simulink model "lab09_observer_controller"  (R2026b)
settings: Solver=VariableStepAuto  StopTime=1.5  RelTol=1e-9
undefined symbols (not defined in the file): A_o, B_o, C_o, D_o, Ki_cont, Km, Kp, tau, Ts, Vdc
libraries: slpidlib x3
settings Model: Creator=Maddo  LastModifiedBy=Maddo
settings DataIOCC: SaveFormat=Structure

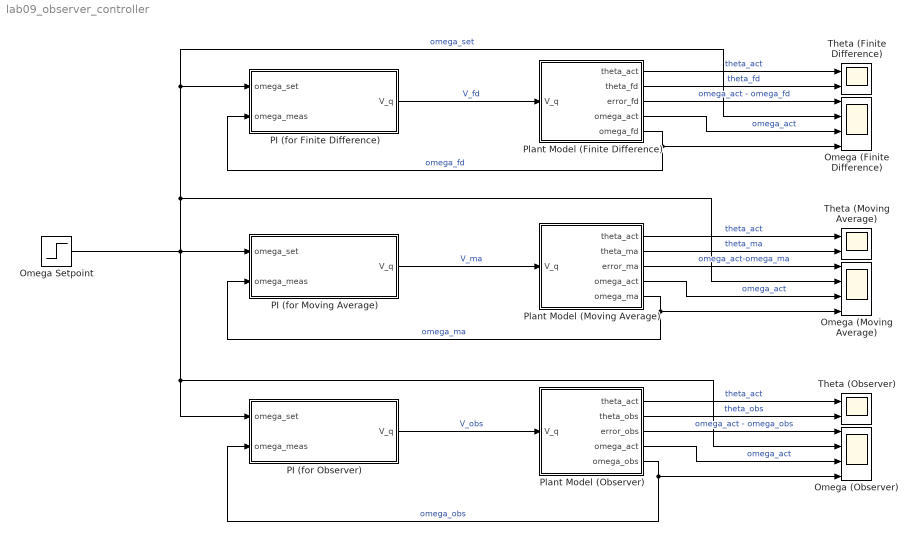
== system lab09_observer_controller ==
  Omega (Finite Difference) : Scope  NumInputPorts=4
      settings: ActiveDisplayYMinimum=-0.40086586035071825  ActiveDisplayYMaximum=0.41815649863978394  DataLoggingVariableName=ScopeData7
  Omega (Moving Average) : Scope  NumInputPorts=4
      settings: ActiveDisplayYMinimum=-1  ActiveDisplayYMaximum=1
  Omega (Observer) : Scope  NumInputPorts=4
      settings: ActiveDisplayYMinimum=-0.10732048180331535  ActiveDisplayYMaximum=0.23324163544595725  DataLoggingVariableName=ScopeData4
  Omega Setpoint : Step  Time=0  FinalValue=omega_set  SampleTime=0
  PI (for Finite Difference) : Subsystem
  PI (for Moving Average) : Subsystem
  PI (for Observer) : Subsystem
  Plant Model (Finite Difference) : Subsystem
  Plant Model (Moving Average) : Subsystem
  Plant Model (Observer) : Subsystem
  Theta (Finite Difference) : Scope  NumInputPorts=2
      settings: ActiveDisplayYMinimum=-1  ActiveDisplayYMaximum=1
  Theta (Moving Average) : Scope  NumInputPorts=2
      settings: ActiveDisplayYMinimum=-1  ActiveDisplayYMaximum=1  DataLoggingVariableName=ScopeData2
  Theta (Observer) : Scope  NumInputPorts=2
      settings: ActiveDisplayYMinimum=1.7677662447249645  ActiveDisplayYMaximum=1.9037236023326192  DataLoggingVariableName=ScopeData5
  wires:
  Plant Model (Finite Difference)/1(theta_act) -> Theta (Finite Difference)/1  "theta_act"
  Plant Model (Finite Difference)/2(theta_fd) -> Theta (Finite Difference)/2  "theta_fd"
  Plant Model (Finite Difference)/4(omega_act) -> Omega (Finite Difference)/3  "omega_act"
  Plant Model (Finite Difference)/5(omega_fd) -> PI (for Finite Difference)/2(omega_meas), Omega (Finite Difference)/4  "omega_fd"
  Plant Model (Finite Difference)/3(error_fd) -> Omega (Finite Difference)/1  "omega_act - omega_fd"
  Plant Model (Moving Average)/3(error_ma) -> Omega (Moving Average)/1  "omega_act-omega_ma"
  Plant Model (Moving Average)/5(omega_ma) -> PI (for Moving Average)/2(omega_meas), Omega (Moving Average)/4  "omega_ma"
  Plant Model (Moving Average)/4(omega_act) -> Omega (Moving Average)/3  "omega_act"
  Plant Model (Moving Average)/2(theta_ma) -> Theta (Moving Average)/2  "theta_ma"
  Plant Model (Moving Average)/1(theta_act) -> Theta (Moving Average)/1  "theta_act"
  Plant Model (Observer)/1(theta_act) -> Theta (Observer)/1  "theta_act"
  Plant Model (Observer)/2(theta_obs) -> Theta (Observer)/2  "theta_obs"
  Plant Model (Observer)/4(omega_act) -> Omega (Observer)/3  "omega_act"
  Plant Model (Observer)/5(omega_obs) -> PI (for Observer)/2(omega_meas), Omega (Observer)/4  "omega_obs"
  Plant Model (Observer)/3(error_obs) -> Omega (Observer)/1  "omega_act - omega_obs"
  Omega Setpoint/1 -> Omega (Moving Average)/2, Omega (Finite Difference)/2, PI (for Finite Difference)/1(omega_set), PI (for Moving Average)/1(omega_set), PI (for Observer)/1(omega_set), Omega (Observer)/2  "omega_set"
  PI (for Finite Difference)/1(V_q) -> Plant Model (Finite Difference)/1(V_q)  "V_fd"
  PI (for Moving Average)/1(V_q) -> Plant Model (Moving Average)/1(V_q)  "V_ma"
  PI (for Observer)/1(V_q) -> Plant Model (Observer)/1(V_q)  "V_obs"

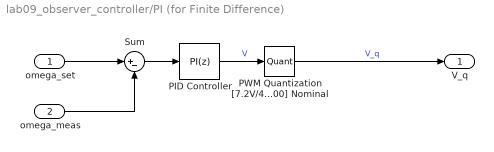
== system lab09_observer_controller/PI (for Finite Difference) ==
  omega_set : Inport
  omega_meas : Inport  Port=2
  PID Controller : slpidlib/PID Controller  Controller=PI  Form=Parallel  TimeDomain=Discrete-time  UseExternalTs=off  SampleTime=Ts  IntegratorMethod=Forward Euler  FilterMethod=Forward Euler  ControllerParametersSource=internal  P=Kp  I=Ki_cont  UseKiTs=off  D=0  UseExternalDerivativeSource=off  N=100  UseFilter=on  TunerSelectOption=Transfer Function Based (PID Tuner App)  InitialConditionSource=internal  InitialConditionForIntegrator=0  InitialConditionForFilter=0  DifferentiatorICPrevScaledInput=0  ExternalReset=none  TrackingMode=off  Kt=1  LimitOutput=on  SatLimitsSource=internal  UpperSaturationLimit=Vdc  LowerSaturationLimit=-Vdc  LinearizeAsGain=on  AntiWindupMode=clamping  Kb=1  LimitIntegrator=off  UpperIntegratorSaturationLimit=inf  LowerIntegratorSaturationLimit=-inf  POutMin=[]  POutMax=[]  IOutMin=[]  IOutMax=[]  DOutMin=[]  DOutMax=[]  NOutMin=[]  NOutMax=[]  SumOutMin=[]  SumOutMax=[]  SaturationOutMin=[]  SaturationOutMax=[]  PParamMin=[]  PParamMax=[]  IParamMin=[]  IParamMax=[]  DParamMin=[]  DParamMax=[]  NParamMin=[]  NParamMax=[]  KbParamMin=[]  KbParamMax=[]  KtParamMin=[]  KtParamMax=[]  KbOutMin=[]  KbOutMax=[]  KtOutMin=[]  KtOutMax=[]  IntegratorOutMin=[]  IntegratorOutMax=[]  FilterOutMin=[]  FilterOutMax=[]  SumI1OutMin=[]  SumI1OutMax=[]  SumI2OutMin=[]  SumI2OutMax=[]  SumI3OutMin=[]  SumI3OutMax=[]  SumI4OutMin=[]  SumI4OutMax=[]  SumDOutMin=[]  SumDOutMax=[]  DifferentiatorOutMin=[]  DifferentiatorOutMax=[]  FilterDiffOutCoefMin=[]  FilterDiffOutCoefMax=[]  ReciprocalOutMin=[]  ReciprocalOutMax=[]  SumDenOutMin=[]  SumDenOutMax=[]  SumNumOutMin=[]  SumNumOutMax=[]  DivideOutMin=[]  DivideOutMax=[]  UdiffTsProdOutMin=[]  UdiffTsProdOutMax=[]  NTsProdOutMin=[]  NTsProdOutMax=[]  UintegralTsProdOutMin=[]  UintegralTsProdOutMax=[]  UngainTsProdOutMin=[]  UngainTsProdOutMax=[]  ClampingZeroOutDataTypeStr=Inherit: Inherit via back propagation  ClampingZeroOutMin=[]  ClampingZeroOutMax=[]  FilterDenConstantOutDataTypeStr=Inherit: Inherit via back propagation  FilterDenConstantOutMin=[]  FilterDenConstantOutMax=[]  PCopyOutDataTypeStr=Inherit: Inherit via back propagation  PCopyOutMin=[]  PCopyOutMax=[]  NCopyOutDataTypeStr=Inherit: Inherit via back propagation  NCopyOutMin=[]  NCopyOutMax=[]  IntegratorContinuousStateAttributes=''  IntegratorStateMustResolveToSignalObject=off  IntegratorRTWStateStorageClass=Auto  FilterContinuousStateAttributes=''  FilterStateMustResolveToSignalObject=off  FilterRTWStateStorageClass=Auto  ParallelPVariant=InternalParameters  IdealPVariant=Disabled  IVariant=InternalParameters  DVariant=Disabled  IntegratorVariant=Discrete  SatVariant=Enabled  AWVariant=DiscClampingParallel  PCopyVariant=Disabled  TRVariant=Disabled  FdbkBlocksVariant=Forward  IdealPFdbkVariant=Disabled  SatFdbkVariant=Disabled  DerivativeFilterVariant=Disabled  NVariant=Disabled  NCopyVariant=Disabled_SignalSpec  FilterICVariant=Disabled  IntegratorICVariant=InternalICs  ExternalResetVariant=Disabled  TRSumVariant=Passthrough  SumFdbkVariant=Disabled  SumVariant=Sum_PI  TsampFilterVariant=InternalTs  TsampNgainVariant=Passthrough  TsampIntegralVariant=Disabled_SignalSpec  ExternalSaturationOutDataTypeStr=Inherit: Same as second input  DerivativeSourceVariant=Disabled  PreIntVariant=InternalPreInt
  PWM Quantization [7.2V/4000] Nominal : Quantizer  QuantizationInterval=Vdc/4000
  Sum : Sum  Inputs=|+-
  V_q : Outport
  wires:
  Sum/1 -> PID Controller/1
  PWM Quantization [7.2V/4000] Nominal/1 -> V_q/1  "V_q"
  PID Controller/1 -> PWM Quantization [7.2V/4000] Nominal/1  "V"
  omega_set/1 -> Sum/1
  omega_meas/1 -> Sum/2

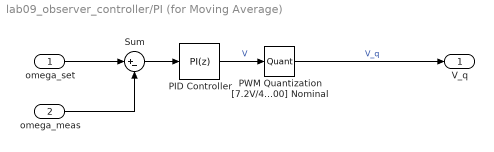
== system lab09_observer_controller/PI (for Moving Average) ==
  omega_set : Inport
  omega_meas : Inport  Port=2
  PID Controller : slpidlib/PID Controller  Controller=PI  Form=Parallel  TimeDomain=Discrete-time  UseExternalTs=off  SampleTime=Ts  IntegratorMethod=Forward Euler  FilterMethod=Forward Euler  ControllerParametersSource=internal  P=Kp  I=Ki_cont  UseKiTs=off  D=0  UseExternalDerivativeSource=off  N=100  UseFilter=on  TunerSelectOption=Transfer Function Based (PID Tuner App)  InitialConditionSource=internal  InitialConditionForIntegrator=0  InitialConditionForFilter=0  DifferentiatorICPrevScaledInput=0  ExternalReset=none  TrackingMode=off  Kt=1  LimitOutput=on  SatLimitsSource=internal  UpperSaturationLimit=Vdc  LowerSaturationLimit=-Vdc  LinearizeAsGain=on  AntiWindupMode=clamping  Kb=1  LimitIntegrator=off  UpperIntegratorSaturationLimit=inf  LowerIntegratorSaturationLimit=-inf  POutMin=[]  POutMax=[]  IOutMin=[]  IOutMax=[]  DOutMin=[]  DOutMax=[]  NOutMin=[]  NOutMax=[]  SumOutMin=[]  SumOutMax=[]  SaturationOutMin=[]  SaturationOutMax=[]  PParamMin=[]  PParamMax=[]  IParamMin=[]  IParamMax=[]  DParamMin=[]  DParamMax=[]  NParamMin=[]  NParamMax=[]  KbParamMin=[]  KbParamMax=[]  KtParamMin=[]  KtParamMax=[]  KbOutMin=[]  KbOutMax=[]  KtOutMin=[]  KtOutMax=[]  IntegratorOutMin=[]  IntegratorOutMax=[]  FilterOutMin=[]  FilterOutMax=[]  SumI1OutMin=[]  SumI1OutMax=[]  SumI2OutMin=[]  SumI2OutMax=[]  SumI3OutMin=[]  SumI3OutMax=[]  SumI4OutMin=[]  SumI4OutMax=[]  SumDOutMin=[]  SumDOutMax=[]  DifferentiatorOutMin=[]  DifferentiatorOutMax=[]  FilterDiffOutCoefMin=[]  FilterDiffOutCoefMax=[]  ReciprocalOutMin=[]  ReciprocalOutMax=[]  SumDenOutMin=[]  SumDenOutMax=[]  SumNumOutMin=[]  SumNumOutMax=[]  DivideOutMin=[]  DivideOutMax=[]  UdiffTsProdOutMin=[]  UdiffTsProdOutMax=[]  NTsProdOutMin=[]  NTsProdOutMax=[]  UintegralTsProdOutMin=[]  UintegralTsProdOutMax=[]  UngainTsProdOutMin=[]  UngainTsProdOutMax=[]  ClampingZeroOutDataTypeStr=Inherit: Inherit via back propagation  ClampingZeroOutMin=[]  ClampingZeroOutMax=[]  FilterDenConstantOutDataTypeStr=Inherit: Inherit via back propagation  FilterDenConstantOutMin=[]  FilterDenConstantOutMax=[]  PCopyOutDataTypeStr=Inherit: Inherit via back propagation  PCopyOutMin=[]  PCopyOutMax=[]  NCopyOutDataTypeStr=Inherit: Inherit via back propagation  NCopyOutMin=[]  NCopyOutMax=[]  IntegratorContinuousStateAttributes=''  IntegratorStateMustResolveToSignalObject=off  IntegratorRTWStateStorageClass=Auto  FilterContinuousStateAttributes=''  FilterStateMustResolveToSignalObject=off  FilterRTWStateStorageClass=Auto  ParallelPVariant=InternalParameters  IdealPVariant=Disabled  IVariant=InternalParameters  DVariant=Disabled  IntegratorVariant=Discrete  SatVariant=Enabled  AWVariant=DiscClampingParallel  PCopyVariant=Disabled  TRVariant=Disabled  FdbkBlocksVariant=Forward  IdealPFdbkVariant=Disabled  SatFdbkVariant=Disabled  DerivativeFilterVariant=Disabled  NVariant=Disabled  NCopyVariant=Disabled_SignalSpec  FilterICVariant=Disabled  IntegratorICVariant=InternalICs  ExternalResetVariant=Disabled  TRSumVariant=Passthrough  SumFdbkVariant=Disabled  SumVariant=Sum_PI  TsampFilterVariant=InternalTs  TsampNgainVariant=Passthrough  TsampIntegralVariant=Disabled_SignalSpec  ExternalSaturationOutDataTypeStr=Inherit: Same as second input  DerivativeSourceVariant=Disabled  PreIntVariant=InternalPreInt
  PWM Quantization [7.2V/4000] Nominal : Quantizer  QuantizationInterval=Vdc/4000
  Sum : Sum  Inputs=|+-
  V_q : Outport
  wires:
  omega_meas/1 -> Sum/2
  omega_set/1 -> Sum/1
  PID Controller/1 -> PWM Quantization [7.2V/4000] Nominal/1  "V"
  PWM Quantization [7.2V/4000] Nominal/1 -> V_q/1  "V_q"
  Sum/1 -> PID Controller/1

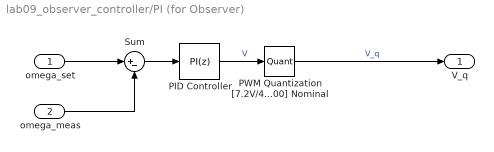
== system lab09_observer_controller/PI (for Observer) ==
  omega_set : Inport
  omega_meas : Inport  Port=2
  PID Controller : slpidlib/PID Controller  Controller=PI  Form=Parallel  TimeDomain=Discrete-time  UseExternalTs=off  SampleTime=Ts  IntegratorMethod=Forward Euler  FilterMethod=Forward Euler  ControllerParametersSource=internal  P=Kp  I=Ki_cont  UseKiTs=off  D=0  UseExternalDerivativeSource=off  N=100  UseFilter=on  TunerSelectOption=Transfer Function Based (PID Tuner App)  InitialConditionSource=internal  InitialConditionForIntegrator=0  InitialConditionForFilter=0  DifferentiatorICPrevScaledInput=0  ExternalReset=none  TrackingMode=off  Kt=1  LimitOutput=on  SatLimitsSource=internal  UpperSaturationLimit=Vdc  LowerSaturationLimit=-Vdc  LinearizeAsGain=on  AntiWindupMode=clamping  Kb=1  LimitIntegrator=off  UpperIntegratorSaturationLimit=inf  LowerIntegratorSaturationLimit=-inf  POutMin=[]  POutMax=[]  IOutMin=[]  IOutMax=[]  DOutMin=[]  DOutMax=[]  NOutMin=[]  NOutMax=[]  SumOutMin=[]  SumOutMax=[]  SaturationOutMin=[]  SaturationOutMax=[]  PParamMin=[]  PParamMax=[]  IParamMin=[]  IParamMax=[]  DParamMin=[]  DParamMax=[]  NParamMin=[]  NParamMax=[]  KbParamMin=[]  KbParamMax=[]  KtParamMin=[]  KtParamMax=[]  KbOutMin=[]  KbOutMax=[]  KtOutMin=[]  KtOutMax=[]  IntegratorOutMin=[]  IntegratorOutMax=[]  FilterOutMin=[]  FilterOutMax=[]  SumI1OutMin=[]  SumI1OutMax=[]  SumI2OutMin=[]  SumI2OutMax=[]  SumI3OutMin=[]  SumI3OutMax=[]  SumI4OutMin=[]  SumI4OutMax=[]  SumDOutMin=[]  SumDOutMax=[]  DifferentiatorOutMin=[]  DifferentiatorOutMax=[]  FilterDiffOutCoefMin=[]  FilterDiffOutCoefMax=[]  ReciprocalOutMin=[]  ReciprocalOutMax=[]  SumDenOutMin=[]  SumDenOutMax=[]  SumNumOutMin=[]  SumNumOutMax=[]  DivideOutMin=[]  DivideOutMax=[]  UdiffTsProdOutMin=[]  UdiffTsProdOutMax=[]  NTsProdOutMin=[]  NTsProdOutMax=[]  UintegralTsProdOutMin=[]  UintegralTsProdOutMax=[]  UngainTsProdOutMin=[]  UngainTsProdOutMax=[]  ClampingZeroOutDataTypeStr=Inherit: Inherit via back propagation  ClampingZeroOutMin=[]  ClampingZeroOutMax=[]  FilterDenConstantOutDataTypeStr=Inherit: Inherit via back propagation  FilterDenConstantOutMin=[]  FilterDenConstantOutMax=[]  PCopyOutDataTypeStr=Inherit: Inherit via back propagation  PCopyOutMin=[]  PCopyOutMax=[]  NCopyOutDataTypeStr=Inherit: Inherit via back propagation  NCopyOutMin=[]  NCopyOutMax=[]  IntegratorContinuousStateAttributes=''  IntegratorStateMustResolveToSignalObject=off  IntegratorRTWStateStorageClass=Auto  FilterContinuousStateAttributes=''  FilterStateMustResolveToSignalObject=off  FilterRTWStateStorageClass=Auto  ParallelPVariant=InternalParameters  IdealPVariant=Disabled  IVariant=InternalParameters  DVariant=Disabled  IntegratorVariant=Discrete  SatVariant=Enabled  AWVariant=DiscClampingParallel  PCopyVariant=Disabled  TRVariant=Disabled  FdbkBlocksVariant=Forward  IdealPFdbkVariant=Disabled  SatFdbkVariant=Disabled  DerivativeFilterVariant=Disabled  NVariant=Disabled  NCopyVariant=Disabled_SignalSpec  FilterICVariant=Disabled  IntegratorICVariant=InternalICs  ExternalResetVariant=Disabled  TRSumVariant=Passthrough  SumFdbkVariant=Disabled  SumVariant=Sum_PI  TsampFilterVariant=InternalTs  TsampNgainVariant=Passthrough  TsampIntegralVariant=Disabled_SignalSpec  ExternalSaturationOutDataTypeStr=Inherit: Same as second input  DerivativeSourceVariant=Disabled  PreIntVariant=InternalPreInt
  PWM Quantization [7.2V/4000] Nominal : Quantizer  QuantizationInterval=Vdc/4000
  Sum : Sum  Inputs=|+-
  V_q : Outport
  wires:
  Sum/1 -> PID Controller/1
  PWM Quantization [7.2V/4000] Nominal/1 -> V_q/1  "V_q"
  PID Controller/1 -> PWM Quantization [7.2V/4000] Nominal/1  "V"
  omega_set/1 -> Sum/1
  omega_meas/1 -> Sum/2

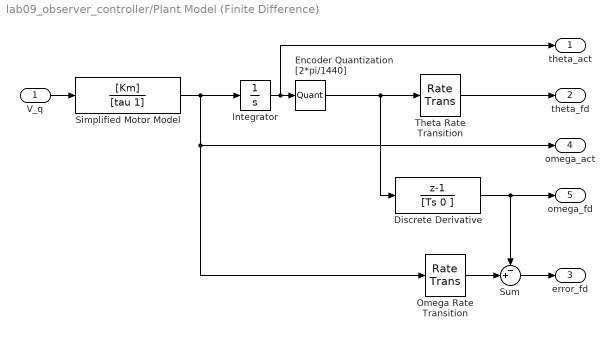
== system lab09_observer_controller/Plant Model (Finite Difference) ==
  V_q : Inport
  Discrete Derivative : DiscreteTransferFcn  Numerator=[1 -1]  Denominator=[Ts 0 ]
  Encoder Quantization [2*pi/1440] : Quantizer  QuantizationInterval=2*pi/1440
  Integrator : Integrator
  Omega Rate Transition : RateTransition  OutPortSampleTime=Ts
  Simplified Motor Model : TransferFcn  Numerator=[Km]  Denominator=[tau 1]
  Sum : Sum  Inputs=-+|
  Theta Rate Transition : RateTransition  OutPortSampleTime=Ts
  theta_act : Outport
  theta_fd : Outport  Port=2
  error_fd : Outport  Port=3
  omega_act : Outport  Port=4
  omega_fd : Outport  Port=5
  wires:
  Integrator/1 -> theta_act/1, Encoder Quantization [2*pi/1440]/1
  Simplified Motor Model/1 -> omega_act/1, Omega Rate Transition/1, Integrator/1
  Encoder Quantization [2*pi/1440]/1 -> Discrete Derivative/1, Theta Rate Transition/1
  Theta Rate Transition/1 -> theta_fd/1
  Discrete Derivative/1 -> Sum/1, omega_fd/1
  V_q/1 -> Simplified Motor Model/1
  Sum/1 -> error_fd/1
  Omega Rate Transition/1 -> Sum/2

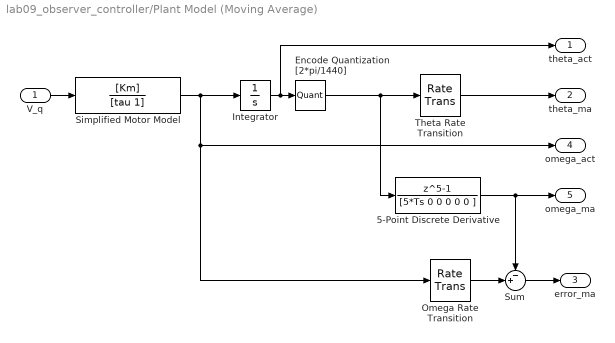
== system lab09_observer_controller/Plant Model (Moving Average) ==
  V_q : Inport
  5-Point Discrete Derivative : DiscreteTransferFcn  Numerator=[1 0 0 0 0 -1]  Denominator=[5*Ts 0 0 0 0 0 ]
  Encode Quantization [2*pi/1440] : Quantizer  QuantizationInterval=2*pi/1440
  Integrator : Integrator
  Omega Rate Transition : RateTransition  OutPortSampleTime=Ts
  Simplified Motor Model : TransferFcn  Numerator=[Km]  Denominator=[tau 1]
  Sum : Sum  Inputs=-+|
  Theta Rate Transition : RateTransition  OutPortSampleTime=Ts
  theta_act : Outport
  theta_ma : Outport  Port=2
  error_ma : Outport  Port=3
  omega_act : Outport  Port=4
  omega_ma : Outport  Port=5
  wires:
  V_q/1 -> Simplified Motor Model/1
  Theta Rate Transition/1 -> theta_ma/1
  Encode Quantization [2*pi/1440]/1 -> 5-Point Discrete Derivative/1, Theta Rate Transition/1
  Integrator/1 -> theta_act/1, Encode Quantization [2*pi/1440]/1
  Simplified Motor Model/1 -> Integrator/1, Omega Rate Transition/1, omega_act/1
  Sum/1 -> error_ma/1
  5-Point Discrete Derivative/1 -> Sum/1, omega_ma/1
  Omega Rate Transition/1 -> Sum/2

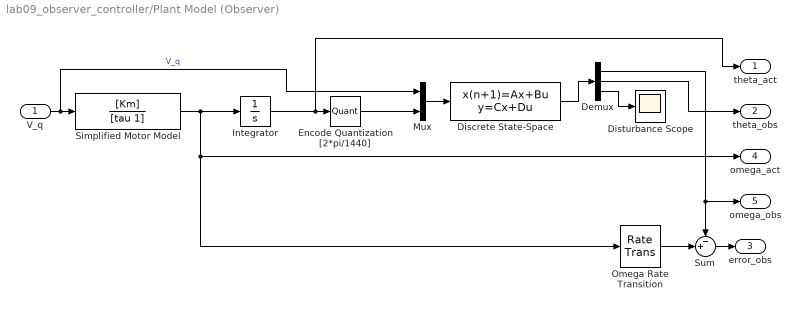
== system lab09_observer_controller/Plant Model (Observer) ==
  V_q : Inport
  Demux : Demux  Outputs=3
  Discrete State-Space : DiscreteStateSpace  A=A_o  B=B_o  C=C_o  D=D_o  SampleTime=Ts
  Disturbance Scope : Scope
      settings: DataLoggingVariableName=ScopeData3
  Encode Quantization [2*pi/1440] : Quantizer  QuantizationInterval=2*pi/1440
  Integrator : Integrator
  Mux : Mux  Inputs=2
  Omega Rate Transition : RateTransition  OutPortSampleTime=Ts
  Simplified Motor Model : TransferFcn  Numerator=[Km]  Denominator=[tau 1]
  Sum : Sum  Inputs=-+|
  theta_act : Outport
  theta_obs : Outport  Port=2
  error_obs : Outport  Port=3
  omega_act : Outport  Port=4
  omega_obs : Outport  Port=5
  wires:
  Integrator/1 -> theta_act/1, Encode Quantization [2*pi/1440]/1
  V_q/1 -> Mux/1, Simplified Motor Model/1  "V_q"
  Mux/1 -> Discrete State-Space/1
  Encode Quantization [2*pi/1440]/1 -> Mux/2
  Discrete State-Space/1 -> Demux/1
  Demux/2 -> theta_obs/1
  Demux/3 -> Disturbance Scope/1
  Simplified Motor Model/1 -> Omega Rate Transition/1, omega_act/1, Integrator/1
  Sum/1 -> error_obs/1
  Demux/1 -> omega_obs/1, Sum/1
  Omega Rate Transition/1 -> Sum/2
